simulink model "Controller"  (R2018b)
settings: configuration reference "control_config" (kept outside this file)
values from neighbouring files (symbols this model uses):
  CONTROL_EXPORT = Simulink.Parameter(CONTROL_EXPORT_VALUE)    [controller_model_init.m]
  CONTROL_PARAM = Simulink.Parameter(CONTROL_PARAM_VALUE)    [controller_model_init.m]
undefined symbols (not defined in the file or in its folder): actuator_cmd, CONTROL_CONST, ControlMode, DiscIntNeverNeededParam, PilotMode, timestamp, VehicleStatus, VTOLState
libraries: simulink x31, FMT_Model_Lib x20
(part 1 of 3)
settings Model: Creator=jc  LastModifiedBy=zouji
settings ConfigSetRef: SourceLocation=Base Workspace

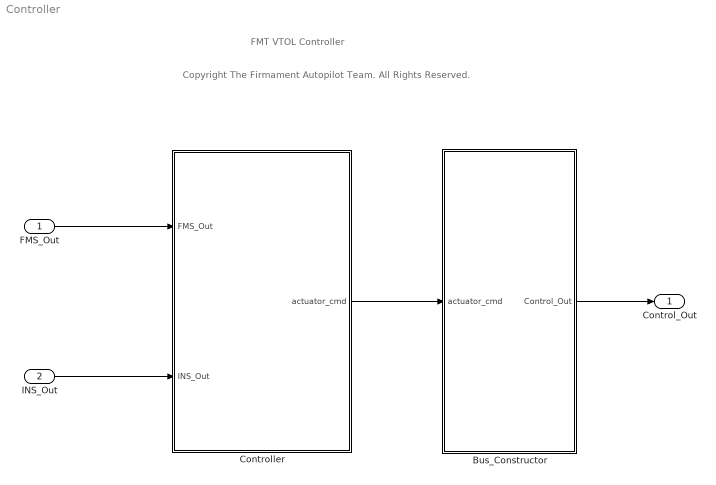
== system Controller ==
  note: Copyright The Firmament Autopilot Team. All Rights Reserved.
  note: FMT VTOL Controller
  FMS_Out : Inport  OutDataTypeStr=Bus: FMS_Out_Bus
  INS_Out : Inport  Port=2  OutDataTypeStr=Bus: INS_Out_Bus
  Bus_Constructor : Subsystem
  Controller : Subsystem
  Control_Out : Outport  OutDataTypeStr=Bus: Control_Out_Bus
  wires:
  FMS_Out/1 -> Controller/1(FMS_Out)
  INS_Out/1 -> Controller/2(INS_Out)
  Controller/1(actuator_cmd) -> Bus_Constructor/1(actuator_cmd)
  Bus_Constructor/1(Control_Out) -> Control_Out/1

== system Controller/Bus_Constructor ==
  actuator_cmd : Inport
  Bus Assignment : BusAssignment  AssignedSignals=actuator_cmd,timestamp
  Constant : Constant  Value=0  OutDataTypeStr=Bus: Control_Out_Bus
  timestamp : Subsystem  mask{sample_time=CONTROL_EXPORT.period}
      mask prompts: sample_time "sample time (ms)"
  Control_Out : Outport
  wires:
  actuator_cmd/1 -> Bus Assignment/2
  Constant/1 -> Bus Assignment/1
  Bus Assignment/1 -> Control_Out/1
  timestamp/1(timestamp_ms) -> Bus Assignment/3

== system Controller/Controller ==
  FMS_Out : Inport
  INS_Out : Inport  Port=2
  ControlFactor : Subsystem
  Data Type Conversion : DataTypeConversion  OutDataTypeStr=single
  Data Type Conversion1 : DataTypeConversion  OutDataTypeStr=single
  FW_Controller : Subsystem  TreatAsAtomicUnit=on
  MC_Controller : Subsystem  TreatAsAtomicUnit=on
  Multiply{,1..3} (4 alike) : Product
  Relay : Relay  OnSwitchValue=0.3  OffSwitchValue=0.1
  Relay1 : Relay  OnSwitchValue=0.3  OffSwitchValue=0.1
  VTOL_Control_Allocation : Subsystem
  actuator_cmd : Outport
  wires:
  INS_Out/1 -> FW_Controller/2(INS_Out), MC_Controller/3(INS_Out)
  FMS_Out/1 -> MC_Controller/4(FMS_Out), ControlFactor/1(FMS_Out), FW_Controller/1(FMS_Out), VTOL_Control_Allocation/1(FMS_Out)
  VTOL_Control_Allocation/1(actuator_cmd) -> actuator_cmd/1
  FW_Controller/3(aux_mc_cmd) -> MC_Controller/1(aux_mc_cmd)
  Relay1/1 -> FW_Controller/Enable, Data Type Conversion/1
  Relay/1 -> MC_Controller/Enable, Data Type Conversion1/1
  FW_Controller/1(fw_torque_cmd) -> Multiply/2
  FW_Controller/2(fw_force_cmd) -> Multiply1/2
  MC_Controller/1(mc_torque_cmd) -> Multiply2/2
  MC_Controller/2(mc_force_cmd) -> Multiply3/2
  Data Type Conversion/1 -> Multiply1/1, Multiply/1
  Multiply/1 -> VTOL_Control_Allocation/2(fw_torque_cmd)
  Multiply1/1 -> VTOL_Control_Allocation/3(fw_force_cmd)
  Multiply2/1 -> VTOL_Control_Allocation/4(mc_torque_cmd)
  Data Type Conversion1/1 -> Multiply3/1, Multiply2/1
  Multiply3/1 -> VTOL_Control_Allocation/5(mc_force_cmd)
  ControlFactor/2(factor_mc) -> Relay/1, MC_Controller/2(factor_mc)  "factor_mc"
  ControlFactor/1(factor_fw) -> Relay1/1, FW_Controller/3(factor_fw)  "factor_fw"

== system Controller/Bus_Constructor/timestamp ==
  Constant : Constant  Value=sample_time
  Data Type Conversion : DataTypeConversion  OutDataTypeStr=uint32
  Discrete-Time Integrator : DiscreteIntegrator  IntegratorMethod=Accumulation: Forward Euler  SampleTime=-1  ICPrevOutput=DiscIntNeverNeededParam  ICPrevScaledInput=DiscIntNeverNeededParam
  timestamp_ms : Outport
  wires:
  Discrete-Time Integrator/1 -> Data Type Conversion/1
  Constant/1 -> Discrete-Time Integrator/1
  Data Type Conversion/1 -> timestamp_ms/1

== system Controller/Controller/ControlFactor ==
  FMS_Out : Inport
  Bus Selector : BusSelector  OutputSignals=ext_state
  Constant : Constant  Value=0  OutDataTypeStr=single
  Constant{1..2,4,7..9} (6 alike) : Constant  OutDataTypeStr=single
  Constant3 : Constant  Value=0.5  OutDataTypeStr=single
  Constant5 : Constant  Value=0.5  OutDataTypeStr=single
  Constant6 : Constant  Value=0  OutDataTypeStr=single
  Demux : Demux  Outputs=2
  First Order LPF1 : FMT_Model_Lib/Filter/First Order LPF  fc=1
      settings: SourceProductName=FMT Toolbox
  First Order LPF3 : FMT_Model_Lib/Filter/First Order LPF  fc=0.5
      settings: SourceProductName=FMT Toolbox
  Multiport Switch : MultiPortSwitch  DataPortOrder=Zero-based contiguous  Inputs=5  zeroidx=on
  Mux{,1..4} (5 alike) : Mux  Inputs=2
  factor_fw : Outport  VectorParamsAs1DForOutWhenUnconnected=on
  factor_mc : Outport  Port=2  VectorParamsAs1DForOutWhenUnconnected=on
  wires:
  Constant1/1 -> Mux/2
  Mux2/1 -> Multiport Switch/4  "Fixwing"
  Constant6/1 -> Mux2/2
  First Order LPF3/1 -> factor_mc/1
  Constant2/1 -> Mux2/1
  Mux/1 -> Multiport Switch/2  "Multicopter"
  Multiport Switch/1 -> Demux/1
  Demux/1 -> First Order LPF1/1
  Demux/2 -> First Order LPF3/1
  Constant/1 -> Mux/1
  Bus Selector/1 -> Multiport Switch/1  "<ext_state>"
  First Order LPF1/1 -> factor_fw/1
  FMS_Out/1 -> Bus Selector/1
  Constant3/1 -> Mux1/1
  Constant4/1 -> Mux1/2
  Mux1/1 -> Multiport Switch/6  "Stall"
  Constant5/1 -> Mux3/1
  Constant7/1 -> Mux3/2
  Mux3/1 -> Multiport Switch/3  "ForwardTrans"
  Mux4/1 -> Multiport Switch/5  "BackwardTrans"
  Constant8/1 -> Mux4/1
  Constant9/1 -> Mux4/2

== system Controller/Controller/FW_Controller ==
  FMS_Out : Inport
  INS_Out : Inport  Port=2
  factor_fw : Inport  Port=3
  Enable : EnablePort  StatesWhenEnabling=reset
  FW_Controller : Subsystem
  Multiply : Product
  Signal_Select : Subsystem
  True_FlySpeed : Subsystem
  fw_torque_cmd : Outport  VectorParamsAs1DForOutWhenUnconnected=on
  fw_force_cmd : Outport  Port=2  VectorParamsAs1DForOutWhenUnconnected=on
  aux_mc_cmd : Outport  Port=3  VectorParamsAs1DForOutWhenUnconnected=on
  wires:
  INS_Out/1 -> True_FlySpeed/1(INS_Out), FW_Controller/2(INS_Out)
  FW_Controller/3(aux_mc_cmd) -> aux_mc_cmd/1
  FMS_Out/1 -> Signal_Select/1(FMS_Out), FW_Controller/1(FMS_Out)
  FW_Controller/1(fw_torque_cmd) -> Signal_Select/2(torque_cmd)  "fw_torque_cmd"
  FW_Controller/2(fw_force_cmd) -> Signal_Select/3(force_cmd)  "fw_force_cmd"
  Signal_Select/1(fw_torque_cmd) -> Multiply/1
  Signal_Select/2(fw_force_cmd) -> fw_force_cmd/1
  factor_fw/1 -> Multiply/2
  Multiply/1 -> fw_torque_cmd/1
  True_FlySpeed/1(VT) -> FW_Controller/3(VT)  "VT"

== system Controller/Controller/MC_Controller ==
  aux_mc_cmd : Inport
  factor_mc : Inport  Port=2
  INS_Out : Inport  Port=3
  FMS_Out : Inport  Port=4
  Enable : EnablePort  StatesWhenEnabling=reset
  Horizontal_Control : Subsystem
  Multiply : Product
  Multiply1 : Product
  Vertical_Control : Subsystem
  mc_torque_cmd : Outport
  mc_force_cmd : Outport  Port=2
  wires:
  INS_Out/1 -> Vertical_Control/2(INS_Out), Horizontal_Control/3(INS_Out)
  FMS_Out/1 -> Vertical_Control/1(FMS_Out), Horizontal_Control/1(FMS_Out)
  aux_mc_cmd/1 -> Horizontal_Control/2(aux_mc_cmd)
  Horizontal_Control/1(torque_cmd_B) -> Multiply/2
  Vertical_Control/1(force_cmd_B) -> Multiply1/2
  factor_mc/1 -> Multiply1/1, Multiply/1
  Multiply/1 -> mc_torque_cmd/1
  Multiply1/1 -> mc_force_cmd/1

== system Controller/Controller/VTOL_Control_Allocation ==
  FMS_Out : Inport
  fw_torque_cmd : Inport  Port=2
  fw_force_cmd : Inport  Port=3
  mc_torque_cmd : Inport  Port=4
  mc_force_cmd : Inport  Port=5
  Bus_Construct : Subsystem
  VTOL_Control_Allocation : Subsystem  Variant=on
      settings: GeneratePreprocessorConditionals=on
  actuator_cmd : Outport  VectorParamsAs1DForOutWhenUnconnected=on
  wires:
  FMS_Out/1 -> VTOL_Control_Allocation/1(FMS_Out)
  Bus_Construct/1(actuator_cmd) -> actuator_cmd/1
  VTOL_Control_Allocation/1(actuator_cmd) -> Bus_Construct/1(vtol_actuator_cmd)
  mc_torque_cmd/1 -> VTOL_Control_Allocation/2(mc_torque_cmd)
  mc_force_cmd/1 -> VTOL_Control_Allocation/3(mc_force_cmd)
  fw_torque_cmd/1 -> VTOL_Control_Allocation/4(fw_torque_cmd)
  fw_force_cmd/1 -> VTOL_Control_Allocation/5(fw_force_cmd)

== system Controller/Controller/FW_Controller/FW_Controller ==
  FMS_Out : Inport
  INS_Out : Inport  Port=2
  VT : Inport  Port=3
  Attitude_Control : Subsystem
  Lateral_Control : Subsystem
  Mux : Mux  Inputs=2
  TECS_Core : Subsystem
  Throttle_Command : Subsystem
  fw_torque_cmd : Outport  VectorParamsAs1DForOutWhenUnconnected=on
  fw_force_cmd : Outport  Port=2  VectorParamsAs1DForOutWhenUnconnected=on
  aux_mc_cmd : Outport  Port=3  VectorParamsAs1DForOutWhenUnconnected=on
  wires:
  INS_Out/1 -> TECS_Core/1(INS_Out), Lateral_Control/2(INS_Out), Attitude_Control/2(INS_Out)
  Lateral_Control/1(phi_cmd) -> Mux/1  "fw_phi_cmd"
  Mux/1 -> Attitude_Control/4(att_cmd)
  TECS_Core/1(fw_pitch_cmd) -> Mux/2  "fw_theta_cmd"
  FMS_Out/1 -> TECS_Core/2(FMS_Out), Throttle_Command/2(FMS_Out), Lateral_Control/1(FMS_Out), Attitude_Control/1(FMS_Out)
  Attitude_Control/1(ang_acc_cmd) -> fw_torque_cmd/1
  VT/1 -> Attitude_Control/3(VT), TECS_Core/3(VT)
  Attitude_Control/2(aux_mc_cmd) -> aux_mc_cmd/1  "aux_mc_cmd"
  TECS_Core/2(fw_throttle_cmd) -> Throttle_Command/1(fw_throttle_cmd)  "fw_throttle_cmd"
  Throttle_Command/1(fw_force_cmd) -> fw_force_cmd/1

== system Controller/Controller/FW_Controller/Signal_Select ==
  FMS_Out : Inport
  torque_cmd : Inport  Port=2
  force_cmd : Inport  Port=3
  Bus Selector1 : BusSelector  OutputSignals=ctrl_mode
  Bus Selector2 : BusSelector  OutputSignals=p_cmd,q_cmd,r_cmd
  Bus Selector3 : BusSelector  OutputSignals=u_cmd
  Constant2 : Constant  Value=0  OutDataTypeStr=single
  Demux : Demux  Outputs=2
  Manual : simulink/Logic and Bit Operations/Compare To Constant  relop===  const=uint8(ControlMode.Manual)  OutDataTypeStr=boolean
  Mux : Mux  Inputs=2
  Mux1 : Mux  Inputs=3
  Mux2 : Mux  Inputs=3
  Mux3 : Mux  Inputs=2
  Switch : Switch  Criteria=u2 > Threshold
  fw_torque_cmd : Outport
  fw_force_cmd : Outport  Port=2
  wires:
  torque_cmd/1 -> Mux/1  "fw_torque_cmd"
  force_cmd/1 -> Mux/2  "fw_force_cmd"
  Bus Selector1/1 -> Manual/1  "<ctrl_mode>"
  Manual/1 -> Switch/2
  Mux/1 -> Switch/3
  Bus Selector3/1 -> Mux1/1  "<u_cmd>"
  FMS_Out/1 -> Bus Selector2/1, Bus Selector3/1, Bus Selector1/1
  Bus Selector2/3 -> Mux2/3  "<r_cmd>"
  Bus Selector2/1 -> Mux2/1  "<p_cmd>"
  Bus Selector2/2 -> Mux2/2  "<q_cmd>"
  Constant2/1 -> Mux1/3, Mux1/2
  Mux2/1 -> Mux3/1  "fw_torque_cmd"
  Mux1/1 -> Mux3/2  "fw_force_cmd"
  Mux3/1 -> Switch/1
  Switch/1 -> Demux/1
  Demux/1 -> fw_torque_cmd/1
  Demux/2 -> fw_force_cmd/1

== system Controller/Controller/FW_Controller/True_FlySpeed ==
  INS_Out : Inport
  Bus Selector2 : BusSelector  OutputSignals=flag
  Bus Selector3 : BusSelector  OutputSignals=airspeed
  First Order LPF3 : FMT_Model_Lib/Filter/First Order LPF  fc=10
      settings: SourceProductName=FMT Toolbox
  Fly_Speed : Subsystem
  Saturation1 : Saturate  UpperLimit=100  LowerLimit=0.1
  Switch : Switch  Criteria=u2 > Threshold
  airspeed_valid : simulink/Logic and Bit Operations/Bitwise Operator  logicop=AND  UseBitMask=on  BitMask=bin2dec('1000000000')  BitMaskRealWorld=Stored Integer
  VT : Outport
  wires:
  INS_Out/1 -> Fly_Speed/1(INS_Out), Bus Selector3/1, Bus Selector2/1
  Bus Selector3/1 -> Switch/1  "<airspeed>"
  Bus Selector2/1 -> airspeed_valid/1  "<flag>"
  First Order LPF3/1 -> VT/1
  Saturation1/1 -> First Order LPF3/1
  Switch/1 -> Saturation1/1
  airspeed_valid/1 -> Switch/2
  Fly_Speed/1(speed) -> Switch/3

== system Controller/Controller/MC_Controller/Horizontal_Control ==
  FMS_Out : Inport
  aux_mc_cmd : Inport  Port=2
  INS_Out : Inport  Port=3
  Attitude_Controller : Subsystem
  Bus Selector : BusSelector  OutputSignals=ctrl_mode
  Compare To Constant : simulink/Logic and Bit Operations/Compare To Constant  relop=>=  const=uint8(ControlMode.POSCTL)  OutDataTypeStr=boolean
  Velocity_Controller : Subsystem
  torque_cmd_B : Outport
  wires:
  Attitude_Controller/1(rate_dot_cmd_B) -> torque_cmd_B/1
  INS_Out/1 -> Velocity_Controller/2(INS_Out), Attitude_Controller/2(INS_Out)
  Velocity_Controller/1(att_cmd_B_rad) -> Attitude_Controller/1(att_cmd_B_rad)
  aux_mc_cmd/1 -> Attitude_Controller/4(aux_mc_cmd)
  FMS_Out/1 -> Bus Selector/1, Attitude_Controller/3(FMS_Out), Velocity_Controller/1(FMS_Out)
  Bus Selector/1 -> Compare To Constant/1  "<ctrl_mode>"
  Compare To Constant/1 -> Velocity_Controller/Enable

== system Controller/Controller/MC_Controller/Vertical_Control ==
  FMS_Out : Inport
  INS_Out : Inport  Port=2
  Bus Selector : BusSelector  OutputSignals=ctrl_mode
  Bus Selector1 : BusSelector  OutputSignals=status
  Compare To Constant : simulink/Logic and Bit Operations/Compare To Constant  relop=>=  const=uint8(ControlMode.ALTCTL)  OutDataTypeStr=boolean
  Delay : Delay  DelayLength=1  InitialCondition=uint8(VehicleStatus.Disarm)
  Signal_Select : Subsystem
  Veloxity_Z_Controller : Subsystem
  force_cmd_B : Outport
  wires:
  INS_Out/1 -> Veloxity_Z_Controller/3(INS_Out)
  Veloxity_Z_Controller/1(throttle_cmd) -> Signal_Select/2(throttle_cmd)
  Signal_Select/1(force_cmd) -> force_cmd_B/1
  Bus Selector/1 -> Compare To Constant/1  "<ctrl_mode>"
  Compare To Constant/1 -> Veloxity_Z_Controller/Enable
  Bus Selector1/1 -> Delay/1  "<status>"
  FMS_Out/1 -> Veloxity_Z_Controller/1(FMS_Out), Signal_Select/1(FMS_Out), Bus Selector/1, Bus Selector1/1
  Delay/1 -> Veloxity_Z_Controller/2(prev_status)

== system Controller/Controller/VTOL_Control_Allocation/Bus_Construct ==
  vtol_actuator_cmd : Inport
  Constant : Constant  Value=zeros(7,1)  VectorParams1D=off  OutDataTypeStr=uint16
  Mux : Mux  Inputs=2
  Reshape : Reshape  OutputDimensionality=Column vector (2-D)  OutputDimensions=[16,1]
  actuator_cmd : Outport  VectorParamsAs1DForOutWhenUnconnected=on
  wires:
  Reshape/1 -> actuator_cmd/1
  Constant/1 -> Mux/2
  Mux/1 -> Reshape/1
  vtol_actuator_cmd/1 -> Mux/1

== system Controller/Controller/VTOL_Control_Allocation/VTOL_Control_Allocation ==
  note: 1) Add Subsystem or Model blocks as valid variant choices.
      | 2) You cannot connect blocks at this level. At simulation, connectivity is automatically
      | determined, based on the active variant and port name matching.
  FMS_Out : Inport
  mc_torque_cmd : Inport  Port=2
  mc_force_cmd : Inport  Port=3
  fw_torque_cmd : Inport  Port=4
  fw_force_cmd : Inport  Port=5
  VTOL1 : Subsystem  TreatAsAtomicUnit=on  VariantControl=AIRFRAME==1
      mask Display: image('.\figures\vtol_1.png');
  VTOL2 : Subsystem  TreatAsAtomicUnit=on  VariantControl=AIRFRAME==2
      mask Display: image('.\figures\vtol_2.png');
  actuator_cmd : Outport

== system Controller/Controller/FW_Controller/FW_Controller/Attitude_Control ==
  FMS_Out : Inport
  INS_Out : Inport  Port=2
  VT : Inport  Port=3
  att_cmd : Inport  Port=4
  Innerloop_Rate_Control : Subsystem
  Outloop_Angle_Control : Subsystem
  ang_acc_cmd : Outport
  aux_mc_cmd : Outport  Port=2
  wires:
  INS_Out/1 -> Outloop_Angle_Control/3(INS_Out), Innerloop_Rate_Control/3(INS_Out)
  FMS_Out/1 -> Outloop_Angle_Control/4(FMS_Out), Innerloop_Rate_Control/2(FMS_Out)
  Innerloop_Rate_Control/1(rate_dot_cmd) -> ang_acc_cmd/1
  att_cmd/1 -> Outloop_Angle_Control/1(att_cmd)
  VT/1 -> Innerloop_Rate_Control/4(VT), Outloop_Angle_Control/2(VT)
  Outloop_Angle_Control/1(fw_euler_rate_cmd) -> aux_mc_cmd/1, Innerloop_Rate_Control/1(fw_euler_rate_cmd)

== system Controller/Controller/FW_Controller/FW_Controller/Lateral_Control ==
  FMS_Out : Inport
  INS_Out : Inport  Port=2
  Atan : Trigonometry  Operator=atan
  Bus Selector : BusSelector  OutputSignals=ay_cmd
  Saturation : Saturate  UpperLimit=CONTROL_PARAM.FW_ROLL_PITCH_CMD_LIM  LowerLimit=-CONTROL_PARAM.FW_ROLL_PITCH_CMD_LIM
  TD : Subsystem
  Terminator : Terminator
  g_force : Gain  Gain=1/9.81
  phi_cmd : Outport
  wires:
  FMS_Out/1 -> Bus Selector/1
  Bus Selector/1 -> TD/1(v)  "<ay_cmd>"
  g_force/1 -> Atan/1
  Atan/1 -> Saturation/1  "phi_cmd"
  INS_Out/1 -> Terminator/1
  Saturation/1 -> phi_cmd/1
  TD/1(v1) -> g_force/1

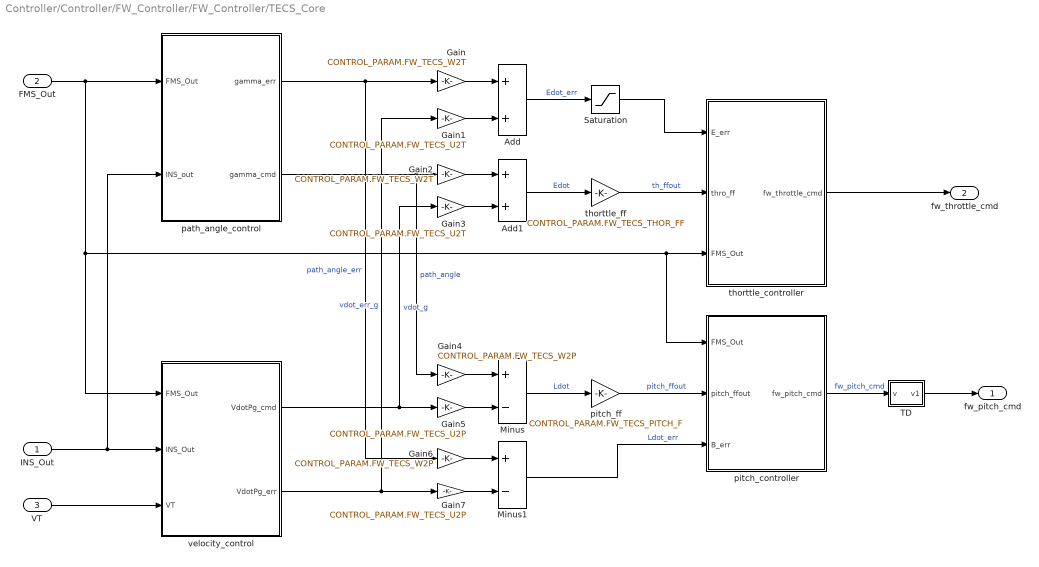
== system Controller/Controller/FW_Controller/FW_Controller/TECS_Core ==
  INS_Out : Inport
  FMS_Out : Inport  Port=2
  VT : Inport  Port=3
  Add : Sum
  Add1 : Sum
  Gain : Gain  Gain=CONTROL_PARAM.FW_TECS_W2T
  Gain1 : Gain  Gain=CONTROL_PARAM.FW_TECS_U2T
  Gain2 : Gain  Gain=CONTROL_PARAM.FW_TECS_W2T
  Gain3 : Gain  Gain=CONTROL_PARAM.FW_TECS_U2T
  Gain4 : Gain  Gain=CONTROL_PARAM.FW_TECS_W2P
  Gain5 : Gain  Gain=CONTROL_PARAM.FW_TECS_U2P
  Gain6 : Gain  Gain=CONTROL_PARAM.FW_TECS_W2P
  Gain7 : Gain  Gain=CONTROL_PARAM.FW_TECS_U2P
  Minus : Sum  Inputs=+-
  Minus1 : Sum  Inputs=+-
  Saturation : Saturate
  TD : Subsystem
  path_angle_control : Subsystem
  pitch_controller : Subsystem
  pitch_ff : Gain  Gain=CONTROL_PARAM.FW_TECS_PITCH_F
  thorttle_controller : Subsystem
  thorttle_ff : Gain  Gain=CONTROL_PARAM.FW_TECS_THOR_FF
  velocity_control : Subsystem
  fw_pitch_cmd : Outport
  fw_throttle_cmd : Outport  Port=2
  wires:
  INS_Out/1 -> path_angle_control/2(INS_out), velocity_control/2(INS_Out)
  path_angle_control/1(gamma_err) -> Gain/1, Gain6/1  "path_angle_err"
  velocity_control/2(VdotPg_err) -> Gain7/1, Gain1/1  "vdot_err_g"
  velocity_control/1(VdotPg_cmd) -> Gain5/1, Gain3/1  "vdot_g"
  path_angle_control/2(gamma_cmd) -> Gain4/1, Gain2/1  "path_angle"
  Minus/1 -> pitch_ff/1  "Ldot"
  Add1/1 -> thorttle_ff/1  "Edot"
  thorttle_ff/1 -> thorttle_controller/2(thro_ff)  "th_ffout"
  pitch_ff/1 -> pitch_controller/2(pitch_ffout)  "pitch_ffout"
  Add/1 -> Saturation/1  "Edot_err"
  Minus1/1 -> pitch_controller/3(B_err)  "Ldot_err"
  Gain4/1 -> Minus/1
  Gain/1 -> Add/1
  Gain1/1 -> Add/2
  thorttle_controller/1(fw_throttle_cmd) -> fw_throttle_cmd/1
  Gain6/1 -> Minus1/1
  Gain7/1 -> Minus1/2
  pitch_controller/1(fw_pitch_cmd) -> TD/1(v)  "fw_pitch_cmd"
  Gain5/1 -> Minus/2
  VT/1 -> velocity_control/3(VT)
  FMS_Out/1 -> velocity_control/1(FMS_Out), pitch_controller/1(FMS_Out), thorttle_controller/3(FMS_Out), path_angle_control/1(FMS_Out)
  Saturation/1 -> thorttle_controller/1(E_err)
  TD/1(v1) -> fw_pitch_cmd/1
  Gain2/1 -> Add1/1
  Gain3/1 -> Add1/2

== system Controller/Controller/FW_Controller/FW_Controller/Throttle_Command ==
  fw_throttle_cmd : Inport
  FMS_Out : Inport  Port=2
  Bias : Bias  Bias=-1
  Bus Selector : BusSelector  OutputSignals=ctrl_mode
  Bus Selector1 : BusSelector  OutputSignals=throttle_cmd
  Compare To Constant : simulink/Logic and Bit Operations/Compare To Constant  relop=<=  const=uint8(ControlMode.Stabilize)  OutDataTypeStr=boolean
  Constant : Constant  Value=0  OutDataTypeStr=single
  Gain : Gain  Gain=1/1000  OutDataTypeStr=single
  Mux1 : Mux  Inputs=3
  Saturation : Saturate  UpperLimit=1  LowerLimit=-1
  Saturation2 : Saturate  UpperLimit=1  LowerLimit=-1
  Switch : Switch  Criteria=u2 > Threshold
  fw_force_cmd : Outport
  wires:
  Saturation2/1 -> fw_force_cmd/1
  Constant/1 -> Mux1/3, Mux1/2
  fw_throttle_cmd/1 -> Saturation/1
  Mux1/1 -> Saturation2/1
  Saturation/1 -> Switch/3
  Compare To Constant/1 -> Switch/2
  FMS_Out/1 -> Bus Selector1/1, Bus Selector/1
  Bus Selector/1 -> Compare To Constant/1  "<ctrl_mode>"
  Bus Selector1/1 -> Gain/1  "<throttle_cmd>"
  Gain/1 -> Bias/1
  Switch/1 -> Mux1/1
  Bias/1 -> Switch/1

== system Controller/Controller/FW_Controller/True_FlySpeed/Fly_Speed ==
  INS_Out : Inport
  Bus Selector2 : BusSelector  OutputSignals=vn,ve,vd
  Bus Selector3 : BusSelector  OutputSignals=quat
  Multiply : Product  Multiplication=Matrix(*)
  Mux : Mux  Inputs=3
  Quaternion To DCM : FMT_Model_Lib/Quaternion/Quaternion To DCM
      settings: SourceProductName=FMT Toolbox
  Selector : Selector  InputPortWidth=3  IndexOptions=Index vector (dialog)  Indices=1  OutputSizes=1
  speed : Outport
  wires:
  Bus Selector3/1 -> Quaternion To DCM/1  "<quat>"
  Multiply/1 -> Selector/1
  Bus Selector2/3 -> Mux/3  "<vd>"
  INS_Out/1 -> Bus Selector3/1, Bus Selector2/1
  Mux/1 -> Multiply/2
  Quaternion To DCM/1 -> Multiply/1
  Bus Selector2/2 -> Mux/2  "<ve>"
  Bus Selector2/1 -> Mux/1  "<vn>"
  Selector/1 -> speed/1

== system Controller/Controller/MC_Controller/Horizontal_Control/Attitude_Controller ==
  att_cmd_B_rad : Inport
  INS_Out : Inport  Port=2
  FMS_Out : Inport  Port=3
  aux_mc_cmd : Inport  Port=4
  Inner_Loop : Subsystem
  Outter_Loop : Subsystem
  rate_dot_cmd_B : Outport
  wires:
  INS_Out/1 -> Inner_Loop/2(INS_Out), Outter_Loop/2(INS_Out)
  FMS_Out/1 -> Inner_Loop/3(FMS_Out), Outter_Loop/3(FMS_Out)
  att_cmd_B_rad/1 -> Outter_Loop/1(att_cmd_rad)
  Outter_Loop/1(euler_rate_cmd_radPs) -> Inner_Loop/1(euler_rate_cmd_radPs)
  Inner_Loop/1(rate_dot_cmd_B) -> rate_dot_cmd_B/1
  aux_mc_cmd/1 -> Inner_Loop/4(aux_mc_cmd)

== system Controller/Controller/MC_Controller/Horizontal_Control/Velocity_Controller ==
  FMS_Out : Inport
  INS_Out : Inport  Port=2
  Enable : EnablePort  StatesWhenEnabling=reset
  Accel_to_Attitude_CMD : Subsystem
  Bus Selector : BusSelector  OutputSignals=reset,ext_state
  Compare To Constant : simulink/Logic and Bit Operations/Compare To Constant  relop=~=  const=uint8(VTOLState.Multicopter)  OutDataTypeStr=boolean
  Error : Subsystem
  Logical Operator : Logic  Operator=OR  AllPortsSameDT=off  OutDataTypeStr=boolean
  PID_Controller : Subsystem
  Signal_Select : Subsystem
  att_cmd_B_rad : Outport
  wires:
  FMS_Out/1 -> Signal_Select/2(FMS_Out), Bus Selector/1, Error/2(FMS_Out)
  PID_Controller/1(accel_cmd_C) -> Signal_Select/1(acc_cmd_in)  "accel_cmd_C_mPs2"
  INS_Out/1 -> Error/1(INS_Out)
  Error/1(uv_err_C_mPs) -> PID_Controller/1(uv_err_C_mPs)
  Accel_to_Attitude_CMD/1(att_cmd_B_rad) -> att_cmd_B_rad/1
  Signal_Select/1(acc_cmd_out) -> Accel_to_Attitude_CMD/1(accel_cmd_C_mPs2)
  Bus Selector/1 -> Logical Operator/1  "<reset>"
  Bus Selector/2 -> Compare To Constant/1  "<ext_state>"
  Logical Operator/1 -> PID_Controller/2(reset)
  Compare To Constant/1 -> Logical Operator/2

== system Controller/Controller/MC_Controller/Vertical_Control/Signal_Select ==
  FMS_Out : Inport
  throttle_cmd : Inport  Port=2
  Bias : Bias  Bias=-1
  Bus Selector1 : BusSelector  OutputSignals=ctrl_mode
  Bus Selector2 : BusSelector  OutputSignals=throttle_cmd
  Compare To Constant : simulink/Logic and Bit Operations/Compare To Constant  relop=<=  const=uint8(ControlMode.Stabilize)  OutDataTypeStr=boolean
  Constant : Constant  Value=0  OutDataTypeStr=single
  Gain : Gain  Gain=1/1000  OutDataTypeStr=single
  Mux : Mux  Inputs=3
  Switch : Switch  Criteria=u2 > Threshold
  force_cmd : Outport
  wires:
  Bus Selector1/1 -> Compare To Constant/1  "<ctrl_mode>"
  Bus Selector2/1 -> Gain/1  "<throttle_cmd>"
  throttle_cmd/1 -> Switch/3
  Constant/1 -> Mux/2, Mux/1
  Compare To Constant/1 -> Switch/2
  Mux/1 -> force_cmd/1
  FMS_Out/1 -> Bus Selector1/1, Bus Selector2/1
  Switch/1 -> Mux/3
  Gain/1 -> Bias/1
  Bias/1 -> Switch/1

== system Controller/Controller/MC_Controller/Vertical_Control/Veloxity_Z_Controller ==
  FMS_Out : Inport
  prev_status : Inport  Port=2
  INS_Out : Inport  Port=3
  Enable : EnablePort  StatesWhenEnabling=reset
  Boosted_Throttle : Subsystem
  Bus Selector : BusSelector  OutputSignals=reset
  Error : Subsystem
  PID_Controller : Subsystem
  Saturation : Saturate  UpperLimit=0.7  LowerLimit=0.3
  Sum : Sum  Inputs=|++
  hover_throttle : Constant  Value=CONTROL_PARAM.MC_HOVER_THRO  OutDataTypeStr=Inherit: Inherit via back propagation
  throttle_cmd : Outport
  wires:
  FMS_Out/1 -> Bus Selector/1, Error/1(FMS_Out)
  INS_Out/1 -> Boosted_Throttle/2(INS_Out), Error/2(INS_Out)
  Boosted_Throttle/1(boosted_thrust) -> Sum/1  "boosted_thrust"
  Error/1(az_cmd_C_mPs2) -> PID_Controller/1(az_cmd_C_mPs2)
  Bus Selector/1 -> PID_Controller/2(reset)  "<reset>"
  PID_Controller/1(thrust_cmd) -> Boosted_Throttle/1(thrust_cmd)
  hover_throttle/1 -> Sum/2
  Sum/1 -> Saturation/1
  Saturation/1 -> throttle_cmd/1
  prev_status/1 -> PID_Controller/3(prev_status)

== system Controller/Controller/VTOL_Control_Allocation/VTOL_Control_Allocation/VTOL1 ==
  FMS_Out : Inport
  mc_torque_cmd : Inport  Port=2
  mc_force_cmd : Inport  Port=3
  fw_torque_cmd : Inport  Port=4
  fw_force_cmd : Inport  Port=5
  Bus Selector : BusSelector  OutputSignals=status
  FW_Control_Allocation : Subsystem  mask{up_limit=CONTROL_PARAM.FW_OUT_MAX, lo_limit=CONTROL_PARAM.FW_OUT_MIN}
      mask prompts: up_limit "Upper Limit"; lo_limit "Lower Limit"
  MC_Control_Allocation : Subsystem  mask{up_lim=CONTROL_PARAM.MC_OUT_MAX, lo_lim=CONTROL_PARAM.MC_OUT_MIN}
      mask prompts: up_lim "Upper Limit"; lo_lim "Lower Limit"
  Mux : Mux  Inputs=2
  Reshape : Reshape  OutputDimensionality=Column vector (2-D)  OutputDimensions=[16,1]
  actuator_cmd_routing : Subsystem
  actuator_cmd : Outport
  wires:
  actuator_cmd_routing/1(cmd_out) -> actuator_cmd/1
  Reshape/1 -> actuator_cmd_routing/1(cmd_in)
  mc_torque_cmd/1 -> MC_Control_Allocation/1(mc_torque_cmd)
  mc_force_cmd/1 -> MC_Control_Allocation/2(mc_force_cmd)
  fw_force_cmd/1 -> FW_Control_Allocation/2(fw_force_cmd)
  FMS_Out/1 -> FW_Control_Allocation/3(FMS_Out), Bus Selector/1
  fw_torque_cmd/1 -> FW_Control_Allocation/1(fw_torque_cmd)
  MC_Control_Allocation/1(mc_actuator_cmd) -> Mux/1
  FW_Control_Allocation/1(fw_actuator_cmd) -> Mux/2
  Mux/1 -> Reshape/1
  Bus Selector/1 -> actuator_cmd_routing/2(status)  "<status>"

== system Controller/Controller/VTOL_Control_Allocation/VTOL_Control_Allocation/VTOL2 ==
  FMS_Out : Inport
  mc_torque_cmd : Inport  Port=2
  mc_force_cmd : Inport  Port=3
  fw_torque_cmd : Inport  Port=4
  fw_force_cmd : Inport  Port=5
  Bus Selector : BusSelector  OutputSignals=status
  FW_Control_Allocation : Subsystem  mask{up_limit=CONTROL_PARAM.FW_OUT_MAX, lo_limit=CONTROL_PARAM.FW_OUT_MIN}
      mask prompts: up_limit "Upper Limit"; lo_limit "Lower Limit"
  MC_Control_Allocation : Subsystem  mask{up_lim=CONTROL_PARAM.MC_OUT_MAX, lo_lim=CONTROL_PARAM.MC_OUT_MIN}
      mask prompts: up_lim "Upper Limit"; lo_lim "Lower Limit"
  Mux : Mux  Inputs=2
  Reshape : Reshape  OutputDimensionality=Column vector (2-D)  OutputDimensions=[16,1]
  actuator_cmd_routing : Subsystem
  actuator_cmd : Outport
  wires:
  actuator_cmd_routing/1(cmd_out) -> actuator_cmd/1
  Reshape/1 -> actuator_cmd_routing/1(cmd_in)
  mc_torque_cmd/1 -> MC_Control_Allocation/1(mc_torque_cmd)
  mc_force_cmd/1 -> MC_Control_Allocation/2(mc_force_cmd)
  fw_force_cmd/1 -> FW_Control_Allocation/2(fw_force_cmd)
  FMS_Out/1 -> FW_Control_Allocation/3(FMS_Out), Bus Selector/1
  fw_torque_cmd/1 -> FW_Control_Allocation/1(fw_torque_cmd)
  MC_Control_Allocation/1(mc_actuator_cmd) -> Mux/1
  FW_Control_Allocation/1(fw_actuator_cmd) -> Mux/2
  Mux/1 -> Reshape/1
  Bus Selector/1 -> actuator_cmd_routing/2(status)  "<status>"

== system Controller/Controller/FW_Controller/FW_Controller/Attitude_Control/Innerloop_Rate_Control ==
  fw_euler_rate_cmd : Inport
  FMS_Out : Inport  Port=2
  INS_Out : Inport  Port=3
  VT : Inport  Port=4
  Add : Sum
  Bus Selector1 : BusSelector  OutputSignals=phi,theta
  Bus Selector2 : BusSelector  OutputSignals=reset
  Bus Selector3 : BusSelector  OutputSignals=p,q,r
  Euler To Angle Rate : FMT_Model_Lib/Math/Euler To Angle Rate
      settings: SourceProductName=FMT Toolbox
  FF : Gain  Gain=CONTROL_PARAM.FW_FF  Multiplication=Matrix(K*u)
  FF_limit : Saturate  UpperLimit=0.3  LowerLimit=-0.3  OutDataTypeStr=single
  Minus2 : Sum  Inputs=+-
  Multiply : Product
  Multiply1 : Product
  Mux : Mux  Inputs=2
  Mux1 : Mux  Inputs=3
  PI_Control : Subsystem
  PI_limit : Saturate  UpperLimit=1  LowerLimit=-1
  PI_scaler : Subsystem
  Saturation1 : Saturate  UpperLimit=1  LowerLimit=-1
  VT_scaler : Subsystem
  rate_dot_cmd : Outport
  wires:
  PI_scaler/1(PI_scale) -> Multiply/1  "PI_scale"
  Multiply1/1 -> FF_limit/1
  FF/1 -> Multiply1/2
  FF_limit/1 -> Add/1  "fw_ff_out"
  VT_scaler/1(FF_scale) -> Multiply1/1  "FF_scale"
  fw_euler_rate_cmd/1 -> Euler To Angle Rate/2  "fw_euler_rate_cmd"
  Multiply/1 -> PI_limit/1
  Euler To Angle Rate/1 -> FF/1, Minus2/1  "fw_rate_cmd_B"
  Mux1/1 -> Minus2/2  "fw_rate_est_B"
  PI_limit/1 -> Add/2  "fw_pi_out"
  Minus2/1 -> PI_Control/1(error)  "fw_rate_err_B"
  Bus Selector2/1 -> PI_Control/2(reset)  "<reset>"
  PI_Control/1(pi_out) -> Multiply/2
  INS_Out/1 -> Bus Selector3/1, Bus Selector1/1
  Bus Selector1/1 -> Mux/1  "<phi>"
  Bus Selector1/2 -> Mux/2  "<theta>"
  Mux/1 -> Euler To Angle Rate/1
  FMS_Out/1 -> Bus Selector2/1
  Bus Selector3/1 -> Mux1/1  "<p>"
  Bus Selector3/2 -> Mux1/2  "<q>"
  Bus Selector3/3 -> Mux1/3  "<r>"
  VT/1 -> PI_scaler/1(VT), VT_scaler/1(VT)
  Add/1 -> Saturation1/1
  Saturation1/1 -> rate_dot_cmd/1

== system Controller/Controller/FW_Controller/FW_Controller/Attitude_Control/Outloop_Angle_Control ==
  att_cmd : Inport
  VT : Inport  Port=2
  INS_Out : Inport  Port=3
  FMS_Out : Inport  Port=4
  Attitude_Controller : Subsystem
  Heading_Controller : Subsystem
  Mux : Mux  Inputs=2
  Reshape : Reshape  OutputDimensionality=Column vector (2-D)
  Signal_Select : Subsystem
  fw_euler_rate_cmd : Outport
  wires:
  FMS_Out/1 -> Heading_Controller/2(FMS_Out), Signal_Select/2(FMS_Out)
  INS_Out/1 -> Attitude_Controller/2(INS_Out)
  att_cmd/1 -> Signal_Select/1(att_cmd_rad)
  Signal_Select/1(fw_att_cmd) -> Heading_Controller/1(fw_att_cmd), Attitude_Controller/1(att_cmd)
  Attitude_Controller/1(phi_theta_rate_cmd) -> Mux/1
  Heading_Controller/1(psi_rate_cmd) -> Mux/2
  Mux/1 -> Reshape/1
  Reshape/1 -> fw_euler_rate_cmd/1
  VT/1 -> Heading_Controller/3(VT)

== system Controller/Controller/FW_Controller/FW_Controller/Lateral_Control/TD ==
  v : Inport
  Integrator : DiscreteIntegrator  SampleTime=-1  ICPrevOutput=DiscIntNeverNeededParam  ICPrevScaledInput=DiscIntNeverNeededParam
  Integrator1 : DiscreteIntegrator  SampleTime=-1  ICPrevOutput=DiscIntNeverNeededParam  ICPrevScaledInput=DiscIntNeverNeededParam
  Subtract : Sum  Inputs=+-
  "fhan " : Subsystem  mask{r0=6*9.806, h0=0.05}
      mask DialogControl ParameterGroupVar Prompt: fhan(v1,v2,r0,h0)
  v1 : Outport
  wires:
  "fhan "/1(fhan) -> Integrator/1
  Subtract/1 -> "fhan "/1(v1)
  Integrator/1 -> Integrator1/1, "fhan "/2(v2)  "v2"
  v/1 -> Subtract/2
  Integrator1/1 -> Subtract/1, v1/1

== system Controller/Controller/FW_Controller/FW_Controller/TECS_Core/TD ==
  v : Inport
  Integrator : DiscreteIntegrator  SampleTime=-1  ICPrevOutput=DiscIntNeverNeededParam  ICPrevScaledInput=DiscIntNeverNeededParam
  Integrator1 : DiscreteIntegrator  SampleTime=-1  ICPrevOutput=DiscIntNeverNeededParam  ICPrevScaledInput=DiscIntNeverNeededParam
  Subtract : Sum  Inputs=+-
  "fhan " : Subsystem  mask{r0=4*pi, h0=0.04}
      mask DialogControl ParameterGroupVar Prompt: fhan(v1,v2,r0,h0)
  v1 : Outport
  wires:
  Integrator1/1 -> v1/1, Subtract/1
  v/1 -> Subtract/2
  Integrator/1 -> Integrator1/1, "fhan "/2(v2)  "v2"
  Subtract/1 -> "fhan "/1(v1)
  "fhan "/1(fhan) -> Integrator/1

== system Controller/Controller/FW_Controller/FW_Controller/TECS_Core/path_angle_control ==
  FMS_Out : Inport
  INS_out : Inport  Port=2
  Flight_Path_Angle : Subsystem
  Fly_Speed : Subsystem
  Subsystem : Subsystem
  Sum : Sum  Inputs=|+-
  Target_Flight_Path_Angle : Subsystem
  gamma_err : Outport
  gamma_cmd : Outport  Port=2
  wires:
  INS_out/1 -> Flight_Path_Angle/1(INS_Out), Fly_Speed/1(INS_Out), Subsystem/1(INS_Out)
  FMS_Out/1 -> Target_Flight_Path_Angle/1(FMS_Out)
  Target_Flight_Path_Angle/1(gamma_sp) -> Sum/1, gamma_cmd/1  "gamma_sp"
  Flight_Path_Angle/1(gamma) -> Sum/2  "gamma"
  Sum/1 -> gamma_err/1
  Subsystem/1(gamma_dir) -> Target_Flight_Path_Angle/2(gamma_dir), Flight_Path_Angle/2(gamma_dir)
  Fly_Speed/1(speed) -> Target_Flight_Path_Angle/3(speed), Flight_Path_Angle/3(speed)

== system Controller/Controller/FW_Controller/FW_Controller/TECS_Core/pitch_controller ==
  FMS_Out : Inport
  pitch_ffout : Inport  Port=2
  B_err : Inport  Port=3
  Add : Sum  Inputs=++++
  Bus Selector : BusSelector  OutputSignals=ext_state
  Compare To Constant : simulink/Logic and Bit Operations/Compare To Constant  relop===  const=uint8(VTOLState.ForwardTrans)  OutDataTypeStr=boolean
  Constant : Constant  Value=0  OutDataTypeStr=single
  D_control : Subsystem
  I_control : Subsystem
  P_control : Gain  Gain=CONTROL_PARAM.FW_TECS_PITCH_P
  Saturation1 : Saturate  UpperLimit=0.3  LowerLimit=-0.3
  Switch : Switch  Criteria=u2 > Threshold
  fw_pitch_cmd : Outport
  wires:
  B_err/1 -> P_control/1, D_control/1(err), I_control/1(err)
  Add/1 -> Switch/3
  D_control/1(d_out) -> Saturation1/1
  P_control/1 -> Add/1  "pitch_pout"
  Saturation1/1 -> Add/3  "pitch_dout"
  I_control/1(i_out) -> Add/2  "pitch_iout"
  FMS_Out/1 -> Bus Selector/1
  Bus Selector/1 -> Compare To Constant/1  "<ext_state>"
  Compare To Constant/1 -> D_control/2(reset), Switch/2, I_control/2(reset)
  pitch_ffout/1 -> Add/4
  Constant/1 -> Switch/1
  Switch/1 -> fw_pitch_cmd/1

== system Controller/Controller/FW_Controller/FW_Controller/TECS_Core/thorttle_controller ==
  E_err : Inport
  thro_ff : Inport  Port=2
  FMS_Out : Inport  Port=3
  " " : DiscreteIntegrator  InitialCondition=0.05  SampleTime=-1  LimitOutput=on  UpperSaturationLimit=1  LowerSaturationLimit=0  ICPrevOutput=DiscIntNeverNeededParam  ICPrevScaledInput=DiscIntNeverNeededParam
  Add4 : Sum  Inputs=+++
  Bus Selector : BusSelector  OutputSignals=ext_state
  Compare To Constant : simulink/Logic and Bit Operations/Compare To Constant  relop===  const=uint8(VTOLState.ForwardTrans)  OutDataTypeStr=boolean
  Constant : Constant  Value=0  OutDataTypeStr=single
  DT Filter : FMT_Model_Lib/Filter/DT Filter  fc=30
      settings: SourceProductName=FMT Toolbox
  Gain : Gain  Gain=CONTROL_PARAM.FW_TECS_THOR_I
  Gain1 : Gain  Gain=CONTROL_PARAM.FW_TECS_THOR_D
  P_control : Gain  Gain=CONTROL_PARAM.FW_TECS_THOR_P
  Saturation1 : Saturate  UpperLimit=0.3  LowerLimit=-0.3
  Sum : Sum  Inputs=++|
  Switch : Switch  Criteria=u2 > Threshold
  fw_throttle_cmd : Outport
  wires:
  Gain1/1 -> Saturation1/1
  P_control/1 -> Add4/1  "th_pout"
  " "/1 -> Sum/1  "th_iout"
  Saturation1/1 -> Add4/2  "th_dout"
  thro_ff/1 -> Add4/3
  FMS_Out/1 -> Bus Selector/1
  Bus Selector/1 -> Compare To Constant/1  "<ext_state>"
  Add4/1 -> Switch/3
  Constant/1 -> Switch/1
  Switch/1 -> Sum/2
  Sum/1 -> fw_throttle_cmd/1
  Gain/1 -> " "/1
  E_err/1 -> Gain/1, P_control/1, DT Filter/1
  DT Filter/1 -> Gain1/1
  Compare To Constant/1 -> DT Filter/2, Switch/2

== system Controller/Controller/FW_Controller/FW_Controller/TECS_Core/velocity_control ==
  note: It may not very correct to use ax as Vdot, but diffirence is not too big
  FMS_Out : Inport
  INS_Out : Inport  Port=2
  VT : Inport  Port=3
  Bus Selector : BusSelector  OutputSignals=u_cmd
  Bus Selector2 : BusSelector  OutputSignals=ax
  Constant : Constant  Value=0  OutDataTypeStr=Inherit: Inherit via back propagation
  DT Filter : FMT_Model_Lib/Filter/DT Filter  fc=1.414
      settings: SourceProductName=FMT Toolbox
  First Order LPF : FMT_Model_Lib/Filter/First Order LPF  fc=5
      settings: SourceProductName=FMT Toolbox
  Gain : Gain  Gain=1/9.81
  Gain1 : Gain  Gain=1/9.81
  Kv : Gain  Gain=CONTROL_PARAM.FW_TECS_VEL_P
  Minus : Sum  Inputs=+-
  Sum : Sum  Inputs=|+-
  Terminator : Terminator
  VdotPg_cmd : Outport
  VdotPg_err : Outport  Port=2
  wires:
  FMS_Out/1 -> Bus Selector/1
  Gain1/1 -> Sum/2  "VdotPg"
  Bus Selector/1 -> Minus/1  "<u_cmd>"
  Gain/1 -> VdotPg_cmd/1, Sum/1  "VdotPg_sp"
  Minus/1 -> Kv/1
  Sum/1 -> VdotPg_err/1  "VdotPg_err"
  VT/1 -> DT Filter/1, Minus/2
  Bus Selector2/1 -> First Order LPF/1  "<ax>"
  INS_Out/1 -> Bus Selector2/1
  First Order LPF/1 -> Terminator/1
  Kv/1 -> Gain/1
  Constant/1 -> DT Filter/2
  DT Filter/1 -> Gain1/1

== system Controller/Controller/MC_Controller/Horizontal_Control/Attitude_Controller/Inner_Loop ==
  euler_rate_cmd_radPs : Inport
  INS_Out : Inport  Port=2
  FMS_Out : Inport  Port=3
  aux_mc_cmd : Inport  Port=4
  ATT_Cmd_Mixer : Subsystem
  Bus Selector : BusSelector  OutputSignals=reset
  Rate_Controller : Subsystem
  rate_dot_cmd_B : Outport
  wires:
  euler_rate_cmd_radPs/1 -> ATT_Cmd_Mixer/2(euler_rate_cmd)
  ATT_Cmd_Mixer/1(rate_cmd_radPs) -> Rate_Controller/1(rate_cmd_radPs)
  Rate_Controller/1(rate_dot_cmd_B) -> rate_dot_cmd_B/1
  Bus Selector/1 -> Rate_Controller/3(reset)  "<reset>"
  INS_Out/1 -> Rate_Controller/2(INS_Out), ATT_Cmd_Mixer/4(INS_Out)
  FMS_Out/1 -> Bus Selector/1, ATT_Cmd_Mixer/1(FMS_Out)
  aux_mc_cmd/1 -> ATT_Cmd_Mixer/3(aux_mc_cmd)

== system Controller/Controller/MC_Controller/Horizontal_Control/Attitude_Controller/Outter_Loop ==
  att_cmd_rad : Inport
  INS_Out : Inport  Port=2
  FMS_Out : Inport  Port=3
  Attitude_Controller : Subsystem
  Signal_Select : Subsystem
  euler_rate_cmd_radPs : Outport
  wires:
  Signal_Select/1(out) -> Attitude_Controller/1(att_cmd_rad)
  FMS_Out/1 -> Signal_Select/2(FMS_Out)
  INS_Out/1 -> Attitude_Controller/2(INS_Out)
  Attitude_Controller/1(euler_rate_cmd_radPs) -> euler_rate_cmd_radPs/1
  att_cmd_rad/1 -> Signal_Select/1(att_cmd_rad)

== system Controller/Controller/MC_Controller/Horizontal_Control/Velocity_Controller/Accel_to_Attitude_CMD ==
  note: Gain to resist
      | air drag
  accel_cmd_C_mPs2 : Inport
  Atan : Trigonometry  Operator=atan
  Divide : Product  Inputs=*/
  Gain1 : Gain  Gain=-1
  Mux : Mux  Inputs=2
  Saturation : Saturate  UpperLimit=CONTROL_PARAM.MC_ROLL_PITCH_CMD_LIM  LowerLimit=-CONTROL_PARAM.MC_ROLL_PITCH_CMD_LIM
  Selector : Selector  InputPortWidth=2  IndexOptions=Index vector (dialog)  Indices=1  OutputSizes=1
  Selector1 : Selector  InputPortWidth=2  IndexOptions=Index vector (dialog)  Indices=2  OutputSizes=1
  g : Constant  Value=9.8055  OutDataTypeStr=single
  gain : Gain  Gain=1.1
  att_cmd_B_rad : Outport
  wires:
  Mux/1 -> gain/1
  gain/1 -> Divide/1
  Atan/1 -> Saturation/1
  g/1 -> Divide/2
  Divide/1 -> Atan/1
  Selector/1 -> Gain1/1
  Selector1/1 -> Mux/1
  accel_cmd_C_mPs2/1 -> Selector/1, Selector1/1
  Gain1/1 -> Mux/2
  Saturation/1 -> att_cmd_B_rad/1

== system Controller/Controller/MC_Controller/Horizontal_Control/Velocity_Controller/Error ==
  INS_Out : Inport
  FMS_Out : Inport  Port=2
  Bus Selector : BusSelector  OutputSignals=u_cmd,v_cmd
  Bus Selector1 : BusSelector  OutputSignals=flag
  Bus_Select : Subsystem
  Compare To Zero : simulink/Logic and Bit Operations/Compare To Zero  relop===  OutDataTypeStr=boolean
  Mux : Mux  Inputs=2
  Sum : Sum  Inputs=|+-
  Switch : Switch  Criteria=u2 > Threshold
  TD : Subsystem
  vel_valid : simulink/Logic and Bit Operations/Bitwise Operator  logicop=AND  UseBitMask=on  BitMask=bin2dec('10000')  BitMaskRealWorld=Stored Integer
  uv_err_C_mPs : Outport
  wires:
  INS_Out/1 -> Bus_Select/1(INS_Out), Bus Selector1/1
  Sum/1 -> uv_err_C_mPs/1  "uv_error_C_mPs"
  vel_valid/1 -> Compare To Zero/1
  Switch/1 -> TD/2(v0)
  Bus Selector/1 -> Mux/1  "<u_cmd>"
  Mux/1 -> Switch/1, TD/1(v)
  Compare To Zero/1 -> Switch/2
  TD/1(v1) -> Sum/1  "uv_cmd_C_mPs"
  Bus Selector1/1 -> vel_valid/1  "<flag>"
  Bus Selector/2 -> Mux/2  "<v_cmd>"
  Bus_Select/1(uv_est_C_mPs) -> Switch/3, Sum/2  "uv_est_C_mPs"
  FMS_Out/1 -> Bus Selector/1

== system Controller/Controller/MC_Controller/Horizontal_Control/Velocity_Controller/PID_Controller ==
  uv_err_C_mPs : Inport
  reset : Inport  Port=2
  Add : Sum  Inputs=+++
  D_Control : Subsystem  mask{kd=CONTROL_PARAM.MC_VEL_XY_D, max_d=CONTROL_PARAM.MC_VEL_XY_D_MAX, min_d=CONTROL_PARAM.MC_VEL_XY_D_MIN}
  I_Control : Subsystem  mask{ki=CONTROL_PARAM.MC_VEL_XY_I, max_i=CONTROL_PARAM.MC_VEL_XY_I_MAX, min_i=CONTROL_PARAM.MC_VEL_XY_I_MIN}
  P_Control : Subsystem  mask{kp=CONTROL_PARAM.MC_VEL_XY_P}
  accel_cmd_C : Outport
  wires:
  uv_err_C_mPs/1 -> P_Control/1(err), I_Control/1(err), D_Control/1(err)
  reset/1 -> I_Control/2(reset), D_Control/2(reset)
  P_Control/1(p_out) -> Add/1  "accel_p_out"
  I_Control/1(i_out) -> Add/2  "accel_i_out"
  D_Control/1(d_out) -> Add/3  "accel_d_out"
  Add/1 -> accel_cmd_C/1

== system Controller/Controller/MC_Controller/Horizontal_Control/Velocity_Controller/Signal_Select ==
  acc_cmd_in : Inport
  FMS_Out : Inport  Port=2
  Bus Selector : BusSelector  OutputSignals=ctrl_mode
  Offboard : simulink/Logic and Bit Operations/Compare To Constant  relop===  const=uint8(ControlMode.Offboard)  OutDataTypeStr=boolean
  Offboard_Signal_Select : Subsystem
  Switch : Switch  Criteria=u2 > Threshold
  acc_cmd_out : Outport
  wires:
  FMS_Out/1 -> Offboard_Signal_Select/1(FMS_Out), Bus Selector/1
  Bus Selector/1 -> Offboard/1  "<ctrl_mode>"
  Offboard/1 -> Switch/2
  Switch/1 -> acc_cmd_out/1
  acc_cmd_in/1 -> Offboard_Signal_Select/2(acc_cmd_in), Switch/3
  Offboard_Signal_Select/1(acc_cmd) -> Switch/1

== system Controller/Controller/MC_Controller/Vertical_Control/Veloxity_Z_Controller/Boosted_Throttle ==
  thrust_cmd : Inport
  INS_Out : Inport  Port=2
  Bus Selector : BusSelector  OutputSignals=phi,theta
  Constant : Constant  OutDataTypeStr=single
  Cos : Trigonometry  Operator=cos
  Cos1 : Trigonometry  Operator=cos
  Divide : Product  Inputs=*/
  Gain : Gain  Gain=2
  Multiply : Product
  Multiply1 : Product  Inputs=3
  Saturation : Saturate  UpperLimit=1  LowerLimit=0
  Saturation1 : Saturate  UpperLimit=1  LowerLimit=0.5
  boosted_thrust : Outport
  wires:
  INS_Out/1 -> Bus Selector/1
  Bus Selector/1 -> Cos/1  "<phi>"
  Bus Selector/2 -> Cos1/1  "<theta>"
  Cos/1 -> Multiply/1
  Cos1/1 -> Multiply/2
  Multiply/1 -> Saturation1/1, Gain/1
  Gain/1 -> Saturation/1
  Saturation/1 -> Multiply1/3  "inverted_factor"
  Constant/1 -> Divide/1
  Divide/1 -> Multiply1/2  "boost_factor"
  Saturation1/1 -> Divide/2
  thrust_cmd/1 -> Multiply1/1
  Multiply1/1 -> boosted_thrust/1

== system Controller/Controller/MC_Controller/Vertical_Control/Veloxity_Z_Controller/Error ==
  FMS_Out : Inport
  INS_Out : Inport  Port=2
  Bus Selector1 : BusSelector  OutputSignals=vd
  Bus Selector2 : BusSelector  OutputSignals=w_cmd,mode
  Compare To Constant : simulink/Logic and Bit Operations/Compare To Constant  relop=>=  const=uint8(PilotMode.Altitude)  OutDataTypeStr=boolean
  Data Type Conversion : DataTypeConversion  OutDataTypeStr=single
  Gain : Gain  Gain=-1  OutDataTypeStr=Inherit: Same as input
  Multiply : Product
  Signal Copy1 : SignalConversion  OverrideOpt=off
  Sum1 : Sum  Inputs=|+-
  Switch : Switch  Criteria=u2 > Threshold
  TD : Subsystem
  az_cmd_C_mPs2 : Outport
  wires:
  INS_Out/1 -> Bus Selector1/1
  Bus Selector2/1 -> Switch/1  "<w_cmd>"
  Bus Selector1/1 -> Signal Copy1/1, Switch/3  "<vd>"
  Gain/1 -> Multiply/2
  Sum1/1 -> Gain/1  "w_error_C_mPs"
  TD/1(v1) -> Sum1/1  "w_cmd_C_mPs"
  FMS_Out/1 -> Bus Selector2/1
  Switch/1 -> TD/1(v)
  Compare To Constant/1 -> Data Type Conversion/1, Switch/2
  Signal Copy1/1 -> Sum1/2  "w_est_C_mPs"
  Bus Selector2/2 -> Compare To Constant/1  "<mode>"
  Data Type Conversion/1 -> Multiply/1
  Multiply/1 -> az_cmd_C_mPs2/1

== system Controller/Controller/MC_Controller/Vertical_Control/Veloxity_Z_Controller/PID_Controller ==
  az_cmd_C_mPs2 : Inport
  reset : Inport  Port=2
  prev_status : Inport  Port=3
  Add : Sum  Inputs=+++
  Compare To Constant : simulink/Logic and Bit Operations/Compare To Constant  relop=<  const=uint8(VehicleStatus.Arm)  OutDataTypeStr=boolean
  D_Control : Subsystem  mask{kd=CONTROL_PARAM.MC_VEL_Z_D, max_d=CONTROL_PARAM.MC_VEL_Z_D_MAX, min_d=CONTROL_PARAM.MC_VEL_Z_D_MIN}
  I_Control : Subsystem  mask{ki=CONTROL_PARAM.MC_VEL_Z_I, max_i=CONTROL_PARAM.MC_VEL_Z_I_MAX, min_i=CONTROL_PARAM.MC_VEL_Z_I_MIN}
  P_Control : Subsystem  mask{kp=CONTROL_PARAM.MC_VEL_Z_P}
  thrust_cmd : Outport
  wires:
  P_Control/1(p_out) -> Add/1  "thrust_p_out"
  I_Control/1(i_out) -> Add/2  "thrust_i_out"
  Add/1 -> thrust_cmd/1
  az_cmd_C_mPs2/1 -> D_Control/1(err), I_Control/1(err), P_Control/1(err)
  D_Control/1(d_out) -> Add/3  "thrust_d_out"
  reset/1 -> I_Control/3(reset), D_Control/2(reset)
  prev_status/1 -> Compare To Constant/1
  Compare To Constant/1 -> I_Control/2(slow_start)

== system Controller/Controller/VTOL_Control_Allocation/VTOL_Control_Allocation/VTOL1/FW_Control_Allocation ==
  fw_torque_cmd : Inport
  fw_force_cmd : Inport  Port=2
  FMS_Out : Inport  Port=3
  Bias : Bias  Bias=1500
  Bias1 : Bias  Bias=CONTROL_PARAM.SERVO1_BIAS
  Bias2 : Bias  Bias=CONTROL_PARAM.SERVO2_BIAS
  Bias3 : Bias  Bias=CONTROL_PARAM.SERVO3_BIAS
  Bias4 : Bias  Bias=CONTROL_PARAM.SERVO4_BIAS
  Data Type Conversion{,1..3} (4 alike) : DataTypeConversion  OutDataTypeStr=uint16
  Demux : Demux
  FW_Effective_Matrix : Subsystem
  Gain1 : Gain  Gain=500  OutDataTypeStr=Inherit: Same as input  ParamDataTypeStr=Inherit: Same as input
  Multiply1 : Product  Multiplication=Matrix(*)  OutDataTypeStr=Inherit: Same as first input
  Mux1 : Mux  Inputs=5
  Saturation : Saturate  UpperLimit=1  LowerLimit=0
  Saturation1 : Saturate  UpperLimit=up_limit  LowerLimit=lo_limit  OutDataTypeStr=uint16
  Saturation5 : Saturate  UpperLimit=1  LowerLimit=-1
  Selector : Selector  InputPortWidth=3  IndexOptions=Index vector (dialog)  Indices=1  OutputSizes=1
  Signal_Select : Subsystem  Commented=on
  fw_throttle_mapping : Subsystem
  fw_actuator_cmd : Outport
  wires:
  Data Type Conversion/1 -> Mux1/2  "aileron_left"
  Gain1/1 -> Bias/1
  Saturation5/1 -> Multiply1/2
  Saturation/1 -> fw_throttle_mapping/1(thrust_cmd)
  Selector/1 -> Saturation/1
  Data Type Conversion1/1 -> Mux1/3  "aileron_right"
  Data Type Conversion3/1 -> Mux1/5  "rudder"
  FW_Effective_Matrix/1(EffecMat) -> Multiply1/1
  fw_force_cmd/1 -> Selector/1
  Data Type Conversion2/1 -> Mux1/4  "elevator"
  Mux1/1 -> Saturation1/1
  Multiply1/1 -> Gain1/1
  fw_torque_cmd/1 -> Saturation5/1
  fw_throttle_mapping/1(throttle_cmd) -> Mux1/1, Signal_Select/1(throttle_cmd_in)  "main_rotor"
  FMS_Out/1 -> Signal_Select/2(FMS_Out)
  Bias/1 -> Demux/1
  Saturation1/1 -> fw_actuator_cmd/1
  Bias2/1 -> Data Type Conversion1/1
  Bias1/1 -> Data Type Conversion/1
  Bias3/1 -> Data Type Conversion2/1
  Bias4/1 -> Data Type Conversion3/1
  Demux/1 -> Bias1/1  "aileron_left"
  Demux/2 -> Bias2/1  "aileron_right"
  Demux/3 -> Bias3/1  "elevator"
  Demux/4 -> Bias4/1  "rudder"

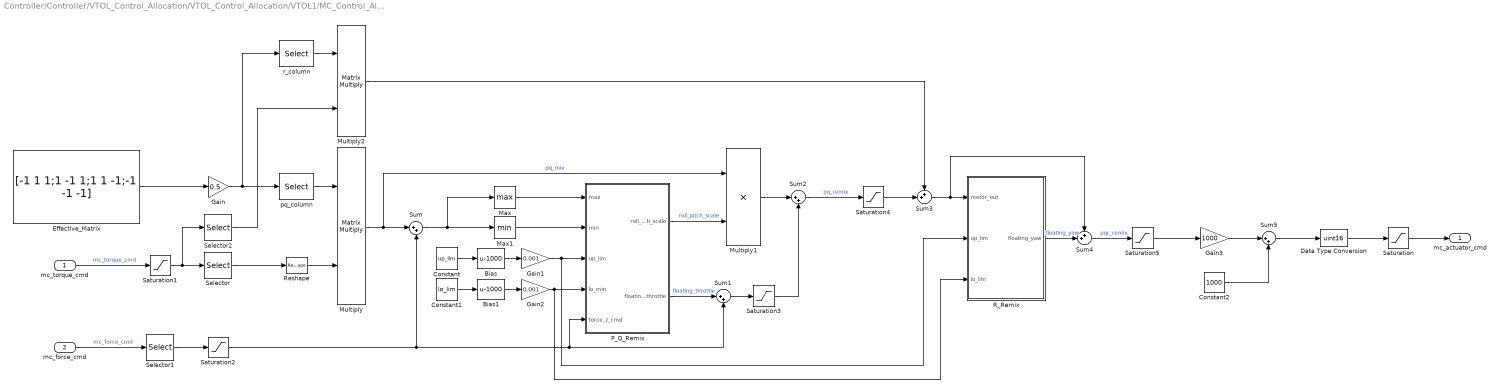
== system Controller/Controller/VTOL_Control_Allocation/VTOL_Control_Allocation/VTOL1/MC_Control_Allocation ==
  mc_torque_cmd : Inport
  mc_force_cmd : Inport  Port=2
  Bias : Bias  Bias=-1000
  Bias1 : Bias  Bias=-1000
  Constant : Constant  Value=up_lim  OutDataTypeStr=single
  Constant1 : Constant  Value=lo_lim  OutDataTypeStr=single
  Constant2 : Constant  Value=1000  OutDataTypeStr=uint32
  Data Type Conversion : DataTypeConversion  OutDataTypeStr=uint16
  Effective_Matrix : Constant  Value=[-1 1 1;1 -1 1;1 1 -1;-1 -1 -1]  OutDataTypeStr=single
  Gain : Gain  Gain=0.5
  Gain1 : Gain  Gain=0.001
  Gain2 : Gain  Gain=0.001
  Gain3 : Gain  Gain=1000  OutDataTypeStr=uint32
  Max : MinMax  Function=max
  Max1 : MinMax
  Multiply : Product  Multiplication=Matrix(*)  OutDataTypeStr=single
  Multiply1 : Product  OutDataTypeStr=single
  Multiply2 : Product  Multiplication=Matrix(*)  OutDataTypeStr=single
  P_Q_Remix : Subsystem
  R_Remix : MATLAB Function  TreatAsAtomicUnit=on
  Reshape : Reshape  OutputDimensionality=Column vector (2-D)
  Saturation : Saturate  UpperLimit=up_lim  LowerLimit=lo_lim
  Saturation1 : Saturate  UpperLimit=1  LowerLimit=-1
  Saturation{2..5} (4 alike) : Saturate  UpperLimit=1  LowerLimit=0
  Selector : Selector  InputPortWidth=3  IndexOptions=Index vector (dialog)  Indices=[1 2]  OutputSizes=1
  Selector1 : Selector  InputPortWidth=3  IndexOptions=Index vector (dialog)  Indices=3  OutputSizes=1
  Selector2 : Selector  InputPortWidth=3  IndexOptions=Index vector (dialog)  Indices=3  OutputSizes=1
  Sum{,1..2,5} (4 alike) : Sum  Inputs=|++
  Sum3 : Sum  Inputs=++|
  Sum4 : Sum  Inputs=++|
  pq_column : Selector  NumberOfDimensions=2  InputPortWidth=3  IndexOptions=Index vector (dialog),Index vector (dialog)  Indices=[1:4],[1 2]  OutputSizes=1,1
  r_column : Selector  NumberOfDimensions=2  InputPortWidth=3  IndexOptions=Index vector (dialog),Index vector (dialog)  Indices=[1:4],3  OutputSizes=1,1
  mc_actuator_cmd : Outport
  wires:
  Multiply/1 -> Multiply1/1, Sum/1  "pq_mix"
  Effective_Matrix/1 -> Gain/1
  mc_force_cmd/1 -> Selector1/1  "mc_force_cmd"
  Sum/1 -> Max/1, Max1/1
  Saturation/1 -> mc_actuator_cmd/1
  Reshape/1 -> Multiply/2
  Selector/1 -> Reshape/1
  Saturation1/1 -> Selector2/1, Selector/1
  Selector1/1 -> Saturation2/1
  pq_column/1 -> Multiply/1
  Max/1 -> P_Q_Remix/1(max)
  Max1/1 -> P_Q_Remix/2(min)
  Gain/1 -> r_column/1, pq_column/1
  P_Q_Remix/2(floating_throttle) -> Sum1/1  "floating_throttle"
  Sum1/1 -> Saturation3/1
  P_Q_Remix/1(roll_pitch_scale) -> Multiply1/2  "roll_pitch_scale"
  Multiply1/1 -> Sum2/1
  Saturation3/1 -> Sum2/2
  Sum2/1 -> Saturation4/1  "pq_remix"
  r_column/1 -> Multiply2/1
  Selector2/1 -> Multiply2/2
  Multiply2/1 -> Sum3/1
  Saturation4/1 -> Sum3/2
  Sum3/1 -> Sum4/1, R_Remix/1(motor_out)
  Constant/1 -> Bias/1
  Constant1/1 -> Bias1/1
  R_Remix/1(floating_yaw) -> Sum4/2  "floating_yaw"
  Sum4/1 -> Saturation5/1  "pqr_remix"
  Data Type Conversion/1 -> Saturation/1
  Bias/1 -> Gain1/1
  Gain1/1 -> P_Q_Remix/3(up_lim), R_Remix/2(up_lim)
  Bias1/1 -> Gain2/1
  Gain2/1 -> P_Q_Remix/4(lo_min), R_Remix/3(lo_lim)
  mc_torque_cmd/1 -> Saturation1/1  "mc_torque_cmd"
  Sum5/1 -> Data Type Conversion/1
  Saturation5/1 -> Gain3/1
  Gain3/1 -> Sum5/1
  Constant2/1 -> Sum5/2
  Saturation2/1 -> Sum1/2, P_Q_Remix/5(force_z_cmd), Sum/2
